simulink model "sf_bus_demo"  (R2025b)
settings: Solver=FixedStepDiscrete  StartTime=0.0  StopTime=10  RelTol=1e-3  EnableMultiTasking=on
PreLoadFcn:
  | load bus_objects;
settings Model: ExtModeAutoUpdateStatusClock=off  Creator=The MathWorks, Inc.  LastModifiedBy=The MathWorks, Inc.
settings SolverCC: AlgebraicLoopSolver=TrustRegion
settings DataIOCC: LimitDataPoints=on  SaveFormat=Structure  SignalLogging=off  SaveTime=off  ReturnWorkspaceOutputs=off
settings OptimizationCC: DefaultParameterBehavior=Inlined  InlineInvariantSignals=on  ReuseModelBlockBuffer=off  ExpressionDepthLimit=2147483647.0  InitFltsAndDblsToZero=on  EfficientMapNaN2IntZero=off  LifeSpan=inf
settings DebuggingCC: SaveWithParameterizedLinksMsg=none  UnderspecifiedInitializationDetection=Classic  MergeDetectMultiDrivingBlocksExec=none  MultiTaskDSMMsg=warning  MultiTaskCondExecSysMsg=none  FcnCallInpInsideContextMsg=warning  UnconnectedInputMsg=warning  UnconnectedOutputMsg=warning  UnconnectedLineMsg=warning  StateNameClashWarn=warning  SFUnexpectedBacktrackingDiag=warning  SFNoUnconditionalDefaultTransitionDiag=warning  SFExecutionAtInitializationDiag=none  ArithmeticOperatorsInVariantConditions=warning
settings HardwareCC: ProdBitPerPointer=32.0  ProdBitPerSizeT=32.0  ProdBitPerPtrDiffT=32.0  ProdLargestAtomicFloat=None  ProdIntDivRoundTo=Undefined  ProdEndianess=Unspecified  ProdWordSize=32.0  ProdHWDeviceType=32-bit Generic
settings ModelReferenceCC: EnableRefExpFcnMdlSchedulingChecks=on  PropagateSignalLabelsOutOfModel=off
settings SFSimCC: SimCustomHeaderCode="#include \"counterbus.h\""  SimUserSources=counterbus.c  SimUseLocalCustomCode=off  SimParseCustomCode=off  CustomCodeUndefinedFunction=UseInterfaceOnly
settings RTWCC: RTWUseLocalCustomCode=off  CustomSource=counterbus.c  GPUComputeCapability=3.5  DLArmComputeVersion=19.05
settings CodeAppCC: StateflowObjectComments=on
settings GRTTargetCC: TargetFcnLib=ansi_tfl_tmw.mat  TargetLangStandard=C89/C90 (ANSI)  CombineOutputUpdateFcns=off  GRTInterface=on
settings ConfigComp: CovMetricSettings=dw  CovSaveCumulativeToWorkspaceVar=on  CovSaveSingleToWorkspaceVar=on  CovExternalEMLEnable=off  CovSFcnEnable=off

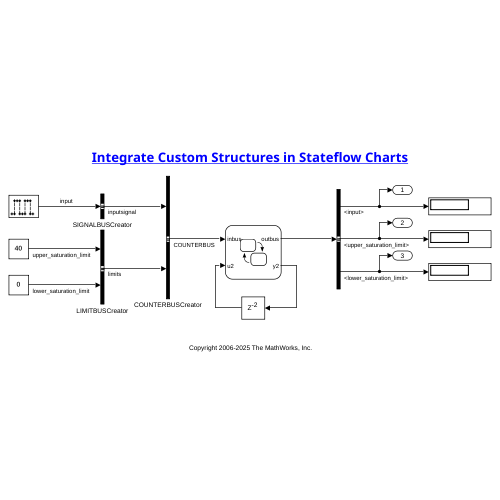
[thumbnail: Simulink's stored preview of the top-level diagram]
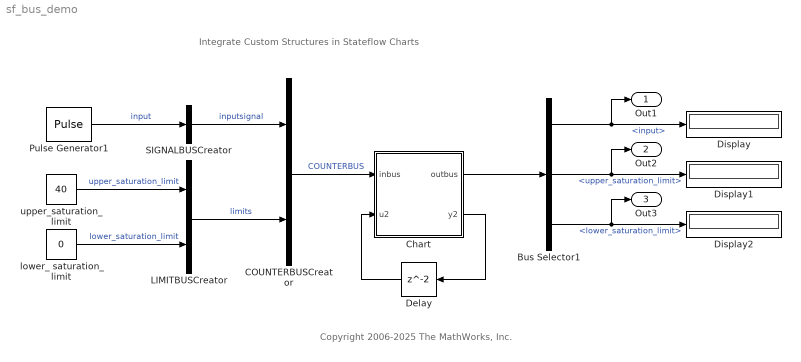
== system sf_bus_demo ==
  note: Copyright 2006-2025 The MathWorks, Inc.
  note: Integrate Custom Structures in Stateflow Charts
  Bus Selector1 : BusSelector  OutputSignals=inputsignal.input,limits.upper_saturation_limit,limits.lower_saturation_limit
  COUNTERBUSCreator : BusCreator  Inputs=2  OutDataTypeStr=Bus: COUNTERBUS  NonVirtualBus=on
  Chart : Stateflow chart  TreatAsAtomicUnit=on
  Delay : Delay
  Display : Display
  Display1 : Display
  Display2 : Display
  LIMITBUSCreator : BusCreator  Inputs=2  OutDataTypeStr=Bus: LIMITBUS  NonVirtualBus=on
  Pulse Generator1 : DiscretePulseGenerator  Amplitude=int32(1)  SampleTime=0.1
  SIGNALBUSCreator : BusCreator  Inputs=1  OutDataTypeStr=Bus: SIGNALBUS  NonVirtualBus=on
  lower_ saturation_ limit : Constant  Value=0  OutDataTypeStr=int32
  upper_saturation_limit : Constant  Value=40  OutDataTypeStr=int32
  Out1 : Outport  VectorParamsAs1DForOutWhenUnconnected=off
  Out2 : Outport  Port=2  VectorParamsAs1DForOutWhenUnconnected=off
  Out3 : Outport  Port=3  VectorParamsAs1DForOutWhenUnconnected=off
  wires:
  upper_saturation_limit/1 -> LIMITBUSCreator/1  "upper_saturation_limit"
  lower_ saturation_ limit/1 -> LIMITBUSCreator/2  "lower_saturation_limit"
  Pulse Generator1/1 -> SIGNALBUSCreator/1  "input"
  LIMITBUSCreator/1 -> COUNTERBUSCreator/2  "limits"
  SIGNALBUSCreator/1 -> COUNTERBUSCreator/1  "inputsignal"
  COUNTERBUSCreator/1 -> Chart/1(inbus)  "COUNTERBUS"
  Chart/2(y2) -> Delay/1
  Delay/1 -> Chart/2(u2)
  Chart/1(outbus) -> Bus Selector1/1
  Bus Selector1/1 -> Display/1, Out1/1  "<input>"
  Bus Selector1/2 -> Display1/1, Out2/1  "<upper_saturation_limit>"
  Bus Selector1/3 -> Display2/1, Out3/1  "<lower_saturation_limit>"

== stateflow chart sf_bus_demo/Chart ==
  (default) -> (junction 4) : {
      | counterbus_struct = inbus;
      | counterbus_struct.inputsignal = inbus.inputsignal;
      |
      | counterbusFcn(&counterbus_struct, u2, &outbus, &y2);
      | }
  data: inbus input Bus: COUNTERBUS size=1; outbus output Bus: COUNTERBUS size=1; u2 input int32; y2 output int32; counterbus_struct local type(inbus)
